simulink model "Es3_simulink"  (R2025b)
settings: Solver=VariableStepAuto  StartTime=0.0  StopTime=10.0  RelTol=1e-3
libraries: simulink x2
settings Model: Creator=fsisa  LastModifiedBy=fsisa

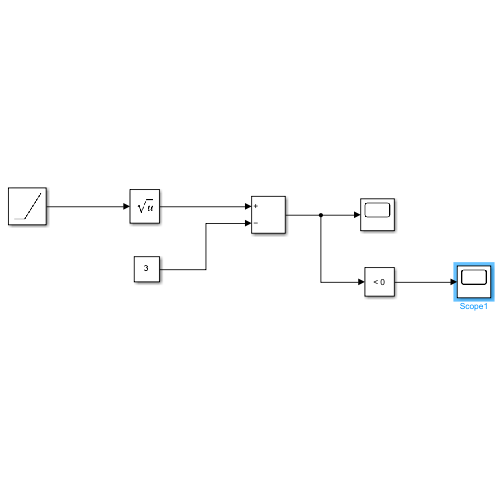
[thumbnail: Simulink's stored preview of the top-level diagram]
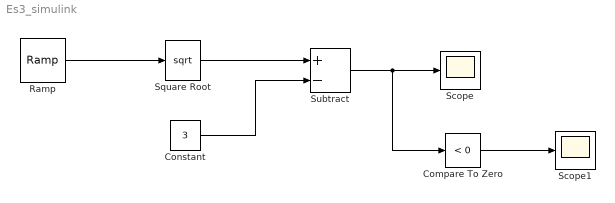
== system Es3_simulink ==
  Compare To Zero : simulink/Logic and Bit Operations/Compare To Zero  relop=<  OutDataTypeStr=boolean
  Constant : Constant  Value=3
  Ramp : simulink/Sources/Ramp  slope=2  start=0  InitialOutput=0
  Scope : Scope
      settings: ActiveDisplayYMinimum=-3.5590169943749475  ActiveDisplayYMaximum=2.0311529493745271
  Scope1 : Scope
      settings: ActiveDisplayYMinimum=-0.12499999999999997  ActiveDisplayYMaximum=1.125
  Square Root : Sqrt
  Subtract : Sum  Inputs=+-
  wires:
  Ramp/1 -> Square Root/1
  Square Root/1 -> Subtract/1
  Constant/1 -> Subtract/2
  Subtract/1 -> Compare To Zero/1, Scope/1
  Compare To Zero/1 -> Scope1/1
